simulink model "APJ6Control"  (R2025b)
settings: Solver=FixedStepAuto  StartTime=0.0  StopTime=10.0  RelTol=1e-3  EnableMultiTasking=on
libraries: simulink x2, slpidlib x1
settings Model: ExtModeTrigDuration=2  Creator=883400  LastModifiedBy=20231207
settings SolverCC: AutoInsertRateTranBlk=on
settings OptimizationCC: EnhancedBackFolding=on  PassReuseOutputArgsAs=Individual arguments  ZeroExternalMemoryAtStartup=off  ZeroInternalMemoryAtStartup=off  MaxStackSize=64  OptimizeBlockOrder=speed  DifferentSizesBufferReuse=on  OptimizationCustomize=off  EfficientTunableParamExpr=on
settings DebuggingCC: ParameterTunabilityLossMsg=error
settings HardwareCC: ProdBitPerPointer=32.0  ProdBitPerSizeT=32.0  ProdBitPerPtrDiffT=32.0  ProdLargestAtomicInteger=Long  ProdLargestAtomicFloat=Double  ProdWordSize=32.0  ProdHWDeviceType=ARM Compatible->ARM Cortex  UseEmbeddedCoderFeatures=off
settings SFSimCC: SimCustomHeaderCode=APJ6_interface.h  MATLABDynamicMemAlloc=off  CustomCodeUndefinedFunction=UseInterfaceOnly
settings RTWCC: SystemTargetFile=ert.tlc  HardwareBoard=Arduino Nano 33 IoT  TemplateMakefile=ert_default_tmf  CustomHeaderCode=APJ6_interface.h  CustomLibrary=apj6_car.a  Toolchain=Arduino ARM  BuildConfiguration=Faster Runs  Description=Embedded Coder
settings CodeAppCC: ForceParamTrailComments=on  IgnoreCustomStorageClasses=off  OperatorAnnotations=on  SimulinkDataObjDesc=on  SFDataObjDesc=on  InsertBlockDesc=on
settings ERTTargetCC: ExtModeTransport=3.0  ExtModeStaticAlloc=on  ExtModeAutomaticAllocSize=off  ExtModeStaticAllocSize=8192.0  ExtModeMexFile=ext_xcp  ExtModeIntrfLevel=Level2 - Open  InlinedParameterPlacement=Hierarchical  SupportContinuousTime=on  SupportNonInlinedSFcns=on  SupportVariableSizeSignals=on

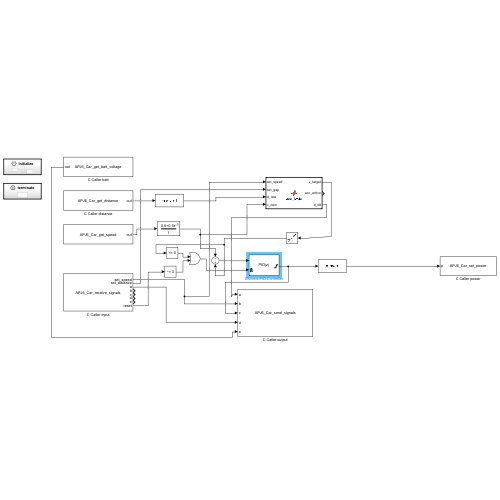
[thumbnail: Simulink's stored preview of the top-level diagram]
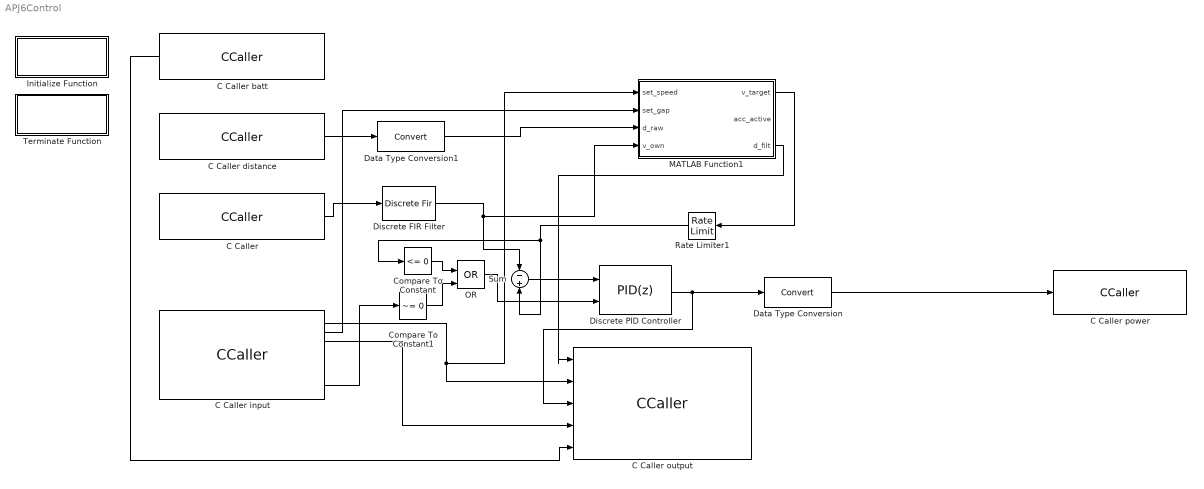
== system APJ6Control ==
  C Caller : CCaller  FunctionName=APJ6_Car_get_speed  PortSpecificationStruct="%)30     .    & (   8    (     @         %    \"     $    !     0         %  0 \"0    $    _    07)G3F%M90  4&]R=$YA;64 4V-O<&4     26YD97@     5'EP90      4VEZ90      27-';&]B86P   X    P    !@    @    $          4    (     0    ,    !         !   P!O=70 #@   #     &    \"     0         !0    @    !     P    $         $  # &]U=  .    .     8    (    !          %    \"     $    &     0         0    !@   $]U='!U=   #@   #@    &    \"     8         !0    @    !     0    $         \"0    @               X    X    !@    @    $          4    (     0    8    !         !     &    <VEN9VQE   .    ,     8    (    !          %    \"     $    !     0         0  $ ,0    X    P    !@    @    ) @        4    (     0    $    !          (  0"
  C Caller batt : CCaller  FunctionName=APJ6_Car_get_batt_voltage  PortSpecificationStruct="%)30     .    & (   8    (     @         %    \"     $    !     0         %  0 \"0    $    _    07)G3F%M90  4&]R=$YA;64 4V-O<&4     26YD97@     5'EP90      4VEZ90      27-';&]B86P   X    P    !@    @    $          4    (     0    ,    !         !   P!O=70 #@   #     &    \"     0         !0    @    !     P    $         $  # &]U=  .    .     8    (    !          %    \"     $    &     0         0    !@   $]U='!U=   #@   #@    &    \"     8         !0    @    !     0    $         \"0    @               X    X    !@    @    $          4    (     0    8    !         !     &    <VEN9VQE   .    ,     8    (    !          %    \"     $    !     0         0  $ ,0    X    P    !@    @    ) @        4    (     0    $    !          (  0"
  C Caller distance : CCaller  FunctionName=APJ6_Car_get_distance  PortSpecificationStruct="%)30     .    & (   8    (     @         %    \"     $    !     0         %  0 \"0    $    _    07)G3F%M90  4&]R=$YA;64 4V-O<&4     26YD97@     5'EP90      4VEZ90      27-';&]B86P   X    P    !@    @    $          4    (     0    ,    !         !   P!O=70 #@   #     &    \"     0         !0    @    !     P    $         $  # &]U=  .    .     8    (    !          %    \"     $    &     0         0    !@   $]U='!U=   #@   #@    &    \"     8         !0    @    !     0    $         \"0    @               X    X    !@    @    $          4    (     0    4    !         !     %    :6YT,S(    .    ,     8    (    !          %    \"     $    !     0         0  $ ,0    X    P    !@    @    ) @        4    (     0    $    !          (  0"
  C Caller input : CCaller  FunctionName=APJ6_Car_receive_signals  PortSpecificationStruct="%)30     .    R T   8    (     @         %    \"     @    !     0         %  0 \"0    $    _    07)G3F%M90  4&]R=$YA;64 4V-O<&4     26YD97@     5'EP90      4VEZ90      27-';&]B86P   X   !     !@    @    $          4    (     0    D    !         !     )    <V5T7W-P965D          X   !     !@    @    $          4    (     0    D    !         !     )    <V5T7W-P965D          X    X    !@    @    $     ...(+4371 chars)"
  C Caller output : CCaller  FunctionName=APJ6_Car_send_signals  PortSpecificationStruct="%)30     .    F @   8    (     @         %    \"     4    !     0         %  0 \"0    $    _    07)G3F%M90  4&]R=$YA;64 4V-O<&4     26YD97@     5'EP90      4VEZ90      27-';&]B86P   X    P    !@    @    $          4    (     0    $    !         !   0!A    #@   #     &    \"     0         !0    @    !     0    $         $  ! &$    .    .     8    (    !          %    \"     $    %     0         0   ...(+2579 chars)"
  C Caller power : CCaller  FunctionName=APJ6_Car_set_power  PortSpecificationStruct="%)30     .    & (   8    (     @         %    \"     $    !     0         %  0 \"0    $    _    07)G3F%M90  4&]R=$YA;64 4V-O<&4     26YD97@     5'EP90      4VEZ90      27-';&]B86P   X    P    !@    @    $          4    (     0    $    !         !   0!P    #@   #     &    \"     0         !0    @    !     0    $         $  ! '     .    .     8    (    !          %    \"     $    %     0         0    !0   $EN<'5T    #@   #@    &    \"     8         !0    @    !     0    $         \"0    @               X    X    !@    @    $          4    (     0    4    !         !     %    :6YT,S(    .    ,     8    (    !          %    \"     $    !     0         0  $ ,0    X    P    !@    @    ) @        4    (     0    $    !          (  0"  SampleTime=0.050
  Compare To Constant : simulink/Logic and Bit Operations/Compare To Constant  relop=<=  const=0  OutDataTypeStr=boolean
  Compare To Constant1 : simulink/Logic and Bit Operations/Compare To Constant  relop=~=  const=0  OutDataTypeStr=boolean
  Data Type Conversion : DataTypeConversion  SaturateOnIntegerOverflow=off  RndMeth=Floor
  Data Type Conversion1 : DataTypeConversion  SaturateOnIntegerOverflow=off  RndMeth=Floor
  Discrete FIR Filter : DiscreteFir
  Discrete PID Controller : slpidlib/PID Controller  Controller=PID  Form=Parallel  TimeDomain=Discrete-time  UseExternalTs=off  SampleTime=0.05  IntegratorMethod=Forward Euler  FilterMethod=Forward Euler  ControllerParametersSource=internal  P=0.15  I=0.25  UseKiTs=off  D=0.5  UseExternalDerivativeSource=off  N=100  UseFilter=on  TunerSelectOption=Transfer Function Based (PID Tuner App)  InitialConditionSource=internal  InitialConditionForIntegrator=0  InitialConditionForFilter=0  DifferentiatorICPrevScaledInput=0  ExternalReset=level  TrackingMode=off  Kt=1  LimitOutput=on  SatLimitsSource=internal  UpperSaturationLimit=170  LowerSaturationLimit=0  LinearizeAsGain=off  AntiWindupMode=clamping  Kb=1  LimitIntegrator=off  UpperIntegratorSaturationLimit=inf  LowerIntegratorSaturationLimit=-inf  POutMin=[]  POutMax=[]  IOutMin=[]  IOutMax=[]  DOutMin=[]  DOutMax=[]  NOutMin=[]  NOutMax=[]  SumOutMin=[]  SumOutMax=[]  SaturationOutMin=[]  SaturationOutMax=[]  PParamMin=[]  PParamMax=[]  IParamMin=[]  IParamMax=[]  DParamMin=[]  DParamMax=[]  NParamMin=[]  NParamMax=[]  KbParamMin=[]  KbParamMax=[]  KtParamMin=[]  KtParamMax=[]  KbOutMin=[]  KbOutMax=[]  KtOutMin=[]  KtOutMax=[]  IntegratorOutMin=[]  IntegratorOutMax=[]  FilterOutMin=[]  FilterOutMax=[]  SumI1OutMin=[]  SumI1OutMax=[]  SumI2OutMin=[]  SumI2OutMax=[]  SumI3OutMin=[]  SumI3OutMax=[]  SumI4OutMin=[]  SumI4OutMax=[]  SumDOutMin=[]  SumDOutMax=[]  DifferentiatorOutMin=[]  DifferentiatorOutMax=[]  FilterDiffOutCoefMin=[]  FilterDiffOutCoefMax=[]  ReciprocalOutMin=[]  ReciprocalOutMax=[]  SumDenOutMin=[]  SumDenOutMax=[]  SumNumOutMin=[]  SumNumOutMax=[]  DivideOutMin=[]  DivideOutMax=[]  UdiffTsProdOutMin=[]  UdiffTsProdOutMax=[]  NTsProdOutMin=[]  NTsProdOutMax=[]  UintegralTsProdOutMin=[]  UintegralTsProdOutMax=[]  UngainTsProdOutMin=[]  UngainTsProdOutMax=[]  ClampingZeroOutDataTypeStr=Inherit: Inherit via back propagation  ClampingZeroOutMin=[]  ClampingZeroOutMax=[]  FilterDenConstantOutDataTypeStr=Inherit: Inherit via back propagation  FilterDenConstantOutMin=[]  FilterDenConstantOutMax=[]  PCopyOutDataTypeStr=Inherit: Inherit via back propagation  PCopyOutMin=[]  PCopyOutMax=[]  NCopyOutDataTypeStr=Inherit: Inherit via back propagation  NCopyOutMin=[]  NCopyOutMax=[]  IntegratorContinuousStateAttributes=''  IntegratorStateMustResolveToSignalObject=off  IntegratorRTWStateStorageClass=Auto  FilterContinuousStateAttributes=''  FilterStateMustResolveToSignalObject=off  FilterRTWStateStorageClass=Auto  ParallelPVariant=InternalParameters  IdealPVariant=Disabled  IVariant=InternalParameters  DVariant=InternalParameters  IntegratorVariant=Discrete  SatVariant=Enabled  AWVariant=DiscClampingParallel  PCopyVariant=Disabled  TRVariant=Disabled  FdbkBlocksVariant=Forward  IdealPFdbkVariant=Disabled  SatFdbkVariant=Disabled  DerivativeFilterVariant=ForwardEulerFilter  NVariant=InternalParameters  NCopyVariant=Disabled  FilterICVariant=InternalICsFilter  IntegratorICVariant=InternalICs  ExternalResetVariant=ExternalReset  TRSumVariant=Passthrough  SumFdbkVariant=Disabled  SumVariant=Sum_PID  TsampFilterVariant=InternalTs  TsampNgainVariant=Passthrough  TsampIntegralVariant=Disabled_SignalSpec  ExternalSaturationOutDataTypeStr=Inherit: Same as second input  DerivativeSourceVariant=ErrorSignal  PreIntVariant=InternalPreInt
      settings: LibrarySourceBlock=simulink/Discrete/Discrete PID Controller
  Initialize Function : Subsystem  TreatAsAtomicUnit=on
  MATLAB Function1 : MATLAB Function  TreatAsAtomicUnit=on
  OR : Logic  Operator=OR  IconShape=distinctive  AllPortsSameDT=off  OutDataTypeStr=boolean
  Rate Limiter1 : RateLimiter  RisingSlewLimit=1500  FallingSlewLimit=-5000  SampleTimeMode=inherited
  Sum : Sum  Inputs=-+
  Terminate Function : Subsystem  TreatAsAtomicUnit=on
  wires:
  C Caller input/3 -> C Caller output/4
  C Caller distance/1 -> Data Type Conversion1/1
  Data Type Conversion1/1 -> MATLAB Function1/3(d_raw)
  C Caller batt/1 -> C Caller output/5
  Discrete PID Controller/1 -> C Caller output/3, Data Type Conversion/1
  Sum/1 -> Discrete PID Controller/1
  C Caller input/1 -> MATLAB Function1/1(set_speed), C Caller output/2
  Data Type Conversion/1 -> C Caller power/1
  C Caller input/8 -> Compare To Constant1/1
  C Caller/1 -> Discrete FIR Filter/1
  Compare To Constant/1 -> OR/1
  Compare To Constant1/1 -> OR/2
  OR/1 -> Discrete PID Controller/2
  C Caller input/2 -> MATLAB Function1/2(set_gap)
  MATLAB Function1/1(v_target) -> Rate Limiter1/1
  MATLAB Function1/3(d_filt) -> C Caller output/1
  Rate Limiter1/1 -> Sum/2, Compare To Constant/1
  Discrete FIR Filter/1 -> Sum/1, MATLAB Function1/4(v_own)

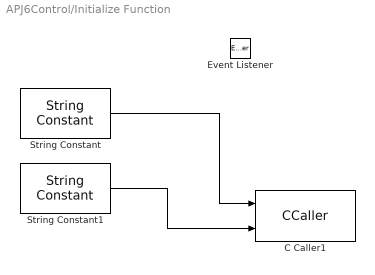
== system APJ6Control/Initialize Function ==
  C Caller1 : CCaller  FunctionName=APJ6_Car_initialize  PortSpecificationStruct="%)30     .    N ,   8    (     @         %    \"     (    !     0         %  0 \"0    $    _    07)G3F%M90  4&]R=$YA;64 4V-O<&4     26YD97@     5'EP90      4VEZ90      27-';&]B86P   X    P    !@    @    $          4    (     0    0    !         !  ! !S<VED#@   #     &    \"     0         !0    @    !    !     $         $  $ '-S:60.    .     8    (    !          %    \"     $    %     0         0    !0   $EN<'5T    #@   #@    &    \"     8         !0    @    !     0    $         \"0    @               X    X    !@    @    $          4    (     0    8    !         !     &    <W1R:6YG   .    ,     8    (    !          %    \"     $    !     0         0  $ ,0    X    P    !@    @    ) @        4    (     0    $    !          (  0      #@   #     &    \"     0         !0    @    !     P    $         $  # '!W9  .    ,     8    (    !          %    \"     $    #     0         0  , <'=D  X    X    !@    @    $          4    (     0    4    !         !     %    26YP=70    .    .     8    (    !@         %    \"     $    !     0         )    \"            / _#@   #@    &    \"     0         !0    @    !    !@    $         $     8   !S=')I;F<   X    P    !@    @    $          4    (     0    $    !         !   0 Q    #@   #     &    \"     D\"        !0    @    !     0    $          @ !"
  Event Listener : EventListener  DisableCoverage=on  EventName=reset
  String Constant : StringConstant  String="\"testcar\""
  String Constant1 : StringConstant  String="\"12345678\""
  wires:
  String Constant1/1 -> C Caller1/2
  String Constant/1 -> C Caller1/1

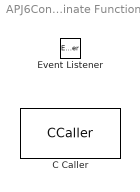
== system APJ6Control/Terminate Function ==
  C Caller : CCaller  FunctionName=APJ6_Car_terminate
  Event Listener : EventListener  DisableCoverage=on  EventType=Terminate  EventName=reset

== matlab function APJ6Control/MATLAB Function1 ==
  data: set_speed input; v_target output; set_gap input; d_raw input; v_own input; acc_active output; d_filt output
function [v_target, acc_active, d_filt] = acc_logic(set_speed, set_gap, d_raw, v_own)
% Adaptive cruise control: outer loop that limits the speed target.

% Work in single precision, whatever type the inputs arrive as
set_speed = single(set_speed);
set_gap   = single(set_gap);
d_raw     = single(d_raw);
v_own     = single(v_own);

Ts      = single(0.05);   % model step (s)
NO_CAR  = single(1400);   % readings at/above this mean "nothing ahead" (sensor reports 1500)
D_STOP  = single(120);    % closer than this: emergency stop
K_GAP   = single(1.0);    % 1/s: how hard to correct the gap error
K_REL   = single(0.3);    % low-pass factor for the closing speed (0..1)
N_SEEN  = 3;              % consecutive valid samples before trusting a target (150 ms)

persistent d1 d2 dprev rel_f count
if isempty(d1)
    d1 = single(1500); d2 = single(1500); dprev = single(1500);
    rel_f = single(0); count = 0;
end

% 1) Median of the last 3 readings removes single-sample spikes
d_med = median([d_raw, d1, d2]);
d2 = d1; d1 = d_raw;

% 2) Only trust an object after it has been seen several samples in a row
if d_med < NO_CAR
    count = min(count + 1, 100);
else
    count = 0;
end
seen = count >= N_SEEN;

% 3) Closing speed from the change in distance, filtered
%    (negative = we are catching up)
if seen && count > N_SEEN
    rel = (d_med - dprev) / Ts;
    rel_f = rel_f + K_REL * (rel - rel_f);
else
    rel_f = single(0);
end
dprev = d_med;

% 4) Gap control: drive at the car ahead's speed, plus a correction for the gap error
gap = set_gap;
if gap <= 0
    gap = single(400);          % default gap if the laptop sends 0
end
v_lead = v_own + rel_f;         % estimated speed of the car ahead
v_acc  = v_lead + K_GAP * (d_med - gap);
v_acc  = max(v_acc, single(0));

% 5) Never go faster than the cruise target; stop if too close
if seen
    v_target = min(set_speed, v_acc);
    if d_med < D_STOP
        v_target = single(0);
    end
else
    v_target = set_speed;
end
acc_active = seen;
d_filt = d_med;
